simulink model "Full_Car_Model"  (R2023b)
settings: Solver=FixedStepAuto  StartTime=0.0  StopTime=t_end_sim  FixedStep=Ts_sim  RelTol=1e-3
values from neighbouring files (symbols this model uses):
  a_b_ref_sat = [ zeros(1,10) ... (first row only)    [A1_Init.m]    (also in C1_MonteCarloAnalysis.m)
  adaptive = 3    [A1_Init.m]    (also in C1_MonteCarloAnalysis.m = 1)
  data = A2_Full_car_model_parameters_4onBoard()    [A1_Init.m]    (also in C1_MonteCarloAnalysis.m)
  Ft_demand_F = [zeros(1,601) 200*ones(1,2400)]./data.R_F    [A1_Init.m]    (also in C1_MonteCarloAnalysis.m)
  Ft_demand_R = [zeros(1,(601-length(l_discr)))              200*ones(1,(2400+length(l_discr)))]./data.R_R    [A1_Init.m]    (also in C1_MonteCarloAnalysis.m)
  handmade_front = strcat(currentPath,'\Road_profiles\height_crg_files\','handmade_step_3cm_singlefunctions.crg')    [A1_Init.m]    (also in C1_MonteCarloAnalysis.m)
  handmade_mu_front = strcat(currentPath,'\Road_profiles\friction_crg_files\','handmade_fric_step_01_singlefunctions.crg')    [A1_Init.m]    (also in C1_MonteCarloAnalysis.m)
  handmade_mu_rear = handmade_mu_front    [A1_Init.m]    (also in C1_MonteCarloAnalysis.m)
  handmade_rear = handmade_front    [A1_Init.m]    (also in C1_MonteCarloAnalysis.m)
  LowLim_Q1 = -10    [A1_Init.m]    (also in C1_MonteCarloAnalysis.m)
  M = N    (= 10)    [A1_Init.m]    (also in C1_MonteCarloAnalysis.m)
  mu_distance = test_distance    [A1_Init.m]    (also in C1_MonteCarloAnalysis.m)
  mu_road = [ones(1,1001), 0.1*ones(1,2000)]    [A1_Init.m]    (also in C1_MonteCarloAnalysis.m)
  N = 10    [A1_Init.m]    (also in C1_MonteCarloAnalysis.m)
  N_iter = 3    [A1_Init.m]    (also in C1_MonteCarloAnalysis.m)
  omega_ini_F_L = x_u_dot_ini_F_L/data.R_F    [A1_Init.m]    (also in C1_MonteCarloAnalysis.m)
  omega_ini_F_R = x_u_dot_ini_R_R/data.R_F    [A1_Init.m]    (also in C1_MonteCarloAnalysis.m)
  omega_ini_R_L = x_u_dot_ini_R_L/data.R_R +2.483*1e-6    [A1_Init.m]    (also in C1_MonteCarloAnalysis.m)
  omega_ini_R_R = x_u_dot_ini_R_R/data.R_R+2.483*1e-6    [A1_Init.m]    (also in C1_MonteCarloAnalysis.m)
  passive = 2    [A1_Init.m]    (also in C1_MonteCarloAnalysis.m)
  Pitch = 0    [A1_Init.m]    (also in C1_MonteCarloAnalysis.m)
  Pitch_dot = 0    [A1_Init.m]    (also in C1_MonteCarloAnalysis.m)
  preview = 2    [A1_Init.m]    (also in C1_MonteCarloAnalysis.m)
  Q1 = 1e6    (= 1000000)    [A1_Init.m]    (also in C1_MonteCarloAnalysis.m)
  Q1_sat = 0    [A1_Init.m]    (also in C1_MonteCarloAnalysis.m)
  Q2 = 1e5    (= 100000)    [A1_Init.m]    (also in C1_MonteCarloAnalysis.m)
  QN1 = 0    [A1_Init.m]    (also in C1_MonteCarloAnalysis.m)
  QN2 = 0    [A1_Init.m]    (also in C1_MonteCarloAnalysis.m)
  R1 = 1e10    (= 10000000000)    [A1_Init.m]    (also in C1_MonteCarloAnalysis.m)
  r1_h0 = 0.99    [A1_Init.m]    (also in C1_MonteCarloAnalysis.m)
  r1_k = 1000    [A1_Init.m]    (also in C1_MonteCarloAnalysis.m)
  r1_max = 11    [A1_Init.m]    (also in C1_MonteCarloAnalysis.m)
  r1_min = -10    [A1_Init.m]    (also in C1_MonteCarloAnalysis.m)
  r2 = 2    [A1_Init.m]    (also in C1_MonteCarloAnalysis.m)
  R2 = 1e2    (= 100)    [A1_Init.m]    (also in C1_MonteCarloAnalysis.m)
  R2_rl = 2    [A1_Init.m]    (also in C1_MonteCarloAnalysis.m)
  road_profile = [zeros(1,801),ones(1,2200)*10*Step_selector]    [A1_Init.m]    (also in C1_MonteCarloAnalysis.m)
  T_distance = test_distance    [A1_Init.m]    (also in C1_MonteCarloAnalysis.m)
  T_hs_ini_F_L = 0    [A1_Init.m]    (also in C1_MonteCarloAnalysis.m)
  T_hs_ini_F_R = 0    [A1_Init.m]    (also in C1_MonteCarloAnalysis.m)
  T_hs_ini_R_L = 0    [A1_Init.m]    (also in C1_MonteCarloAnalysis.m)
  T_hs_ini_R_R = 0    [A1_Init.m]    (also in C1_MonteCarloAnalysis.m)
  test_distance = 0:0.01:30    [A1_Init.m]    (also in C1_MonteCarloAnalysis.m)
  theta_s_ini_F_L = 0    [A1_Init.m]    (also in C1_MonteCarloAnalysis.m)
  theta_s_ini_F_R = 0    [A1_Init.m]    (also in C1_MonteCarloAnalysis.m)
  theta_s_ini_R_L = 0    [A1_Init.m]    (also in C1_MonteCarloAnalysis.m)
  theta_s_ini_R_R = 0    [A1_Init.m]    (also in C1_MonteCarloAnalysis.m)
  theta_w_ini_F_L = -1.056*1e-2    (= -0.01056)    [A1_Init.m]    (also in C1_MonteCarloAnalysis.m)
  theta_w_ini_R_L = -1.056*1e-2    (= -0.01056)    [A1_Init.m]    (also in C1_MonteCarloAnalysis.m)
  Ts = 1e-3*[0 5 10 15 20 25 30 40 60 80 100]    [A1_Init.m]    (also in C1_MonteCarloAnalysis.m)
  w1_h0 = 0.0008    [A1_Init.m]    (also in C1_MonteCarloAnalysis.m)
  w1_k = 5000    [A1_Init.m]    (also in C1_MonteCarloAnalysis.m)
  w1_max = 9    [A1_Init.m]    (also in C1_MonteCarloAnalysis.m)
  w1_min = -10    [A1_Init.m]    (also in C1_MonteCarloAnalysis.m)
  w1_sat = 0.085    [A1_Init.m]    (also in C1_MonteCarloAnalysis.m)
  w2_h0 = 2    [A1_Init.m]    (also in C1_MonteCarloAnalysis.m)
  w2_inc = 0.05    [A1_Init.m]    (also in C1_MonteCarloAnalysis.m)
  w2_k = 10    [A1_Init.m]    (also in C1_MonteCarloAnalysis.m)
  w2_max = 5.3    [A1_Init.m]    (also in C1_MonteCarloAnalysis.m)
  w2_min = -10    [A1_Init.m]    (also in C1_MonteCarloAnalysis.m)
  Wmat_NMPC_init = [W(1,:) W(2,:) W(3,:) W(4,:)]    [A1_Init.m]    (also in C1_MonteCarloAnalysis.m)
  WNmat_NMPC_init = [WN(1,:) WN(2,:)]    [A1_Init.m]    (also in C1_MonteCarloAnalysis.m)
  X_0 = [z_b_dot_ini z_b_ini z_u_dot_ini_F_L z_u_ini_F_L x_b_dot_ini x_b_ini x_u_dot_ini_F_L x_u_ini_F_L          omega_ini_F_L theta_w_ini_F_L omega_ini_F_L theta_s_ini_F_L torque_ini_F_L]    [A1_Init.m]    (also in C1_MonteCarloAnalysis.m)
  x_b_dot_ini = speed_ini/3.6    (= 11.1111111111)    [A1_Init.m]    (also in C1_MonteCarloAnalysis.m)
  x_b_ini = data.b+pos_ini    [A1_Init.m]    (also in C1_MonteCarloAnalysis.m)
  x_u_dot_ini_F_L = speed_ini/3.6 - 1.125*1e-4    (= 11.1109986111)    [A1_Init.m]    (also in C1_MonteCarloAnalysis.m)
  x_u_dot_ini_F_R = speed_ini/3.6 - 1.125*1e-4    (= 11.1109986111)    [A1_Init.m]    (also in C1_MonteCarloAnalysis.m)
  x_u_dot_ini_R_L = speed_ini/3.6 - 1.125*1e-4    (= 11.1109986111)    [A1_Init.m]    (also in C1_MonteCarloAnalysis.m)
  x_u_dot_ini_R_R = speed_ini/3.6 - 1.125*1e-4    (= 11.1109986111)    [A1_Init.m]    (also in C1_MonteCarloAnalysis.m)
  x_u_ini_F_L = data.a+data.b+pos_ini    [A1_Init.m]    (also in C1_MonteCarloAnalysis.m)
  x_u_ini_F_R = data.a+data.b+pos_ini    [A1_Init.m]    (also in C1_MonteCarloAnalysis.m)
  x_u_ini_R_L = pos_ini    (= 0)    [A1_Init.m]    (also in C1_MonteCarloAnalysis.m)
  x_u_ini_R_R = pos_ini    (= 0)    [A1_Init.m]    (also in C1_MonteCarloAnalysis.m)
  z_b_dot_ini = 0    [A1_Init.m]    (also in C1_MonteCarloAnalysis.m)
  z_b_ini = 0    [A1_Init.m]    (also in C1_MonteCarloAnalysis.m)
  z_u_dot_ini_F_L = 0    [A1_Init.m]    (also in C1_MonteCarloAnalysis.m)
  z_u_dot_ini_F_R = 0    [A1_Init.m]    (also in C1_MonteCarloAnalysis.m)
  z_u_dot_ini_R_L = 0    [A1_Init.m]    (also in C1_MonteCarloAnalysis.m)
  z_u_dot_ini_R_R = 0    [A1_Init.m]    (also in C1_MonteCarloAnalysis.m)
  z_u_ini_F_L = 0    [A1_Init.m]    (also in C1_MonteCarloAnalysis.m)
  z_u_ini_F_R = 0    [A1_Init.m]    (also in C1_MonteCarloAnalysis.m)
  z_u_ini_R_L = 0    [A1_Init.m]    (also in C1_MonteCarloAnalysis.m)
  z_u_ini_R_R = 0    [A1_Init.m]    (also in C1_MonteCarloAnalysis.m)
undefined symbols (not defined in the file or in its folder): Delay_step, road_with_noise
libraries: mfswift_library x8, rllib x4, simulink x4
(part 7 of 7)

== matlab function Full_Car_Model/CONTROLLER REAR LEFT/Rule based/MATLAB Function3 ==
  data: flag input; mu_prev input; W output; M parameter; r1_min parameter; r1_max parameter; r1_k parameter; r1_h0 parameter
function W = fcn(flag, mu_prev,M, r1_min, r1_max, r1_k, r1_h0)
h=0; 

x2 = linspace(0, 1, M+1);    
exp_growth = exp(1 * x2) - 1;  

perc = exp_growth; 
perc = perc / sum(perc);

for i=1:M+1
    h=h+mu_prev(i)*perc(i);
end

W=r1_min+(r1_max-r1_min)/(1+exp(r1_k*(abs(h)-r1_h0)));

if not(flag)
    W = r1_min;
end

== matlab function Full_Car_Model/PLANT MODEL WITH MF-SWIFT/4 ON-BOARD POWERTRAIN - FRONT/LEFT HALF SHAFT TORQUES WITH BACKLASH/MATLAB Function2 ==
  data: f1 output; delta_theta input; backlash_F4 input
function f1 = f1_with_backlash(delta_theta, backlash_F4)

if delta_theta < -backlash_F4
    f1 = 1;
else
    f1 = 0;
end

== matlab function Full_Car_Model/PLANT MODEL WITH MF-SWIFT/4 ON-BOARD POWERTRAIN - FRONT/LEFT HALF SHAFT TORQUES WITH BACKLASH/MATLAB Function3 ==
  data: f2 output; delta_theta input; backlash_F4 input
function f2 = f2_with_backlash(delta_theta, backlash_F4)

if delta_theta > backlash_F4
    f2 = 1;
else
    f2 = 0;
end

== matlab function Full_Car_Model/PLANT MODEL WITH MF-SWIFT/4 ON-BOARD POWERTRAIN - FRONT/SHAFT EQUATIONS ==
  data: theta_s_ddot_L output; T_t_L input; theta_s_ddot_R output; T_hs_L input; T_t_R input; T_hs_R input; data parameter
function [theta_s_ddot_L, theta_s_ddot_R] = open_differential_equations(T_t_L, T_hs_L, T_t_R, T_hs_R, data)

theta_s_ddot_L = (T_t_L - T_hs_L) / data.J_eq_F4;
theta_s_ddot_R = (T_t_R - T_hs_R) / data.J_eq_F4;

== matlab function Full_Car_Model/PLANT MODEL WITH MF-SWIFT/4 ON-BOARD POWERTRAIN - FRONT/RIGHT HALF SHAFT TORQUES WITH BACKLASH/MATLAB Function2 ==
  data: f1 output; delta_theta input; backlash_F4 input
function f1 = f1_with_backlash(delta_theta, backlash_F4)

if delta_theta < -backlash_F4
    f1 = 1;
else
    f1 = 0;
end

== matlab function Full_Car_Model/PLANT MODEL WITH MF-SWIFT/4 ON-BOARD POWERTRAIN - FRONT/RIGHT HALF SHAFT TORQUES WITH BACKLASH/MATLAB Function3 ==
  data: f2 output; delta_theta input; backlash_F4 input
function f2 = f2_with_backlash(delta_theta, backlash_F4)

if delta_theta > backlash_F4
    f2 = 1;
else
    f2 = 0;
end

== matlab function Full_Car_Model/PLANT MODEL WITH MF-SWIFT/4 ON-BOARD POWERTRAIN - REAR/LEFT HALF SHAFT TORQUES WITH BACKLASH/MATLAB Function2 ==
  data: f1 output; delta_theta input; backlash_R4 input
function f1 = f1_with_backlash(delta_theta, backlash_R4)

if delta_theta < -backlash_R4
    f1 = 1;
else
    f1 = 0;
end

== matlab function Full_Car_Model/PLANT MODEL WITH MF-SWIFT/4 ON-BOARD POWERTRAIN - REAR/LEFT HALF SHAFT TORQUES WITH BACKLASH/MATLAB Function3 ==
  data: f2 output; delta_theta input; backlash_R4 input
function f2 = f2_with_backlash(delta_theta, backlash_R4)

if delta_theta > backlash_R4
    f2 = 1;
else
    f2 = 0;
end

== matlab function Full_Car_Model/PLANT MODEL WITH MF-SWIFT/4 ON-BOARD POWERTRAIN - REAR/OPEN DIFFERENTIAL EQUATIONS ==
  data: theta_s_ddot_L output; T_t_L input; theta_s_ddot_R output; T_hs_L input; T_t_R input; T_hs_R input; data parameter
function [theta_s_ddot_L, theta_s_ddot_R] = open_differential_equations(T_t_L, T_hs_L, T_t_R, T_hs_R, data)

theta_s_ddot_L = (T_t_L - T_hs_L) / data.J_eq_R4;
theta_s_ddot_R = (T_t_R - T_hs_R) / data.J_eq_R4;

== matlab function Full_Car_Model/PLANT MODEL WITH MF-SWIFT/4 ON-BOARD POWERTRAIN - REAR/RIGHT HALF SHAFT TORQUES WITH BACKLASH/MATLAB Function2 ==
  data: f1 output; delta_theta input; backlash_R4 input
function f1 = f1_with_backlash(delta_theta, backlash_R4)

if delta_theta < -backlash_R4
    f1 = 1;
else
    f1 = 0;
end

== matlab function Full_Car_Model/PLANT MODEL WITH MF-SWIFT/4 ON-BOARD POWERTRAIN - REAR/RIGHT HALF SHAFT TORQUES WITH BACKLASH/MATLAB Function3 ==
  data: f2 output; delta_theta input; backlash_R4 input
function f2 = f2_with_backlash(delta_theta, backlash_R4)

if delta_theta > backlash_R4
    f2 = 1;
else
    f2 = 0;
end

== matlab function Full_Car_Model/PLANT MODEL WITH MF-SWIFT/SUSPENSION MODEL/LONGITUDINAL DYNAMICS/Longitudinal Balance ==
  data: x_b_dot input; Fk_x_R_L input; Fc_x_R_L input; Fk_x_R_R input; Fc_x_R_R input; Fk_x_F_L input; Fc_x_F_L input; Fk_x_F_R input; Fc_x_F_R input; F_x_R_L input; F_x_R_R input; F_x_F_L input; F_x_F_R input; x_b_dot_dot output; x_u_dot_dot_R_L output; x_u_dot_dot_R_R output; x_u_dot_dot_F_L output; x_u_dot_dot_F_R output; data parameter
function [x_b_dot_dot, x_u_dot_dot_R_L, x_u_dot_dot_R_R, x_u_dot_dot_F_L, x_u_dot_dot_F_R] = ...
    fcn(x_b_dot, Fk_x_R_L, Fc_x_R_L, Fk_x_R_R, Fc_x_R_R, Fk_x_F_L, Fc_x_F_L, Fk_x_F_R, Fc_x_F_R, F_x_R_L, F_x_R_R, F_x_F_L, F_x_F_R, data)

F_drag = data.Aero_Coeff*x_b_dot^2;

x_b_dot_dot = (- Fk_x_R_L - Fc_x_R_L - Fk_x_R_R - Fc_x_R_R...
               - Fk_x_F_L - Fc_x_F_L - Fk_x_F_R - Fc_x_F_R...
               - F_drag) / data.m_b;
x_u_dot_dot_R_L = (Fk_x_R_L + Fc_x_R_L + F_x_R_L) / data.m_u_R;
x_u_dot_dot_R_R = (Fk_x_R_R + Fc_x_R_R + F_x_R_R) / data.m_u_R;

x_u_dot_dot_F_L = (Fk_x_F_L + Fc_x_F_L + F_x_F_L) / data.m_u_F;
x_u_dot_dot_F_R = (Fk_x_F_R + Fc_x_F_R + F_x_F_R) / data.m_u_F;

== matlab function Full_Car_Model/CONTROLLER FRONT RIGHT/RL_weights/MATLAB Function ==
  data: w_prev input; h output; M parameter
function h = fcn(w_prev,M)
h=0;   
w1_memo=5;
w_var=zeros(1,M+w1_memo+1);

x1 = linspace(0, 1, w1_memo);         
x2 = linspace(1, 0, M+1); 
exp_growth = exp(1 * x1) - 1;   
exp_decay = exp(1 * x2) - 1;  

perc = [exp_growth, exp_decay]; 
perc = perc / sum(perc);

for i=1:M+w1_memo
    w_var(i)=w_prev(i+1)-w_prev(i); 
    h=h+w_var(i)*perc(i);
end

== matlab function Full_Car_Model/PLANT MODEL WITH MF-SWIFT/SUSPENSION MODEL/ROTATIONAL DYNAMICS/Angular balance ==
  data: Fk_x_R_L input; Fc_x_R_L input; Fk_z_R_L input; Fc_z_R_L input; Fk_x_R_R input; Fc_x_R_R input; Fk_z_R_R input; Fc_z_R_R input; Fk_x_F_L input; Fc_x_F_L input; Fk_z_F_L input; Fc_z_F_L input; Fk_x_F_R input; Fc_x_F_R input; Fk_z_F_R input; Fc_z_F_R input; Mz_AP input; Fu_z_R_L input; Fu_z_R_R input; Fu_z_F_L input; Fu_z_F_R input; pitch_dot_dot output; data parameter
function pitch_dot_dot  ...
    = fcn(Fk_x_R_L, Fc_x_R_L, Fk_z_R_L, Fc_z_R_L, Fk_x_R_R, Fc_x_R_R, Fk_z_R_R, Fc_z_R_R,...
    Fk_x_F_L, Fc_x_F_L, Fk_z_F_L, Fc_z_F_L, Fk_x_F_R, Fc_x_F_R, Fk_z_F_R, Fc_z_F_R,...
    Mz_AP, Fu_z_R_L, Fu_z_R_R, Fu_z_F_L, Fu_z_F_R, data)

pitch_dot_dot = ( (Fk_z_R_L + Fc_z_R_L + Fu_z_R_L + Fk_z_R_R + Fc_z_R_R + Fu_z_R_R)*data.b...
                 -(Fk_z_F_L + Fc_z_F_L + Fu_z_F_L + Fk_z_F_R + Fc_z_F_R + Fu_z_F_R)*data.a...
                 -(Fk_x_R_L + Fc_x_R_L + Fk_x_R_R + Fc_x_R_R + Fk_x_F_L + Fc_x_F_L + Fk_x_F_R + Fc_x_F_R)*data.hg...
                 + Mz_AP)/ (2*data.I_b_y);

== matlab function Full_Car_Model/PLANT MODEL WITH MF-SWIFT/SUSPENSION MODEL/VERTICAL DYNAMICS/Vertical Balance ==
  data: z_b_dot_dot output; z_u_dot_dot_R_L output; z_u_dot_dot_R_R output; Fk_z_R_L input; Fc_z_R_L input; Fk_z_R_R input; Fc_z_R_R input; Fk_z_F_L input; Fc_z_F_L input; Fk_z_F_R input; Fc_z_F_R input; F_z_R_L input; F_z_R_R input; F_z_F_L input; F_z_F_R input; Fu_AP_F input; Fu_AP_R input; Fz_AP input; Fu_z_R_L input; Fu_z_R_R input; Fu_z_F_L input; Fu_z_F_R input; z_u_dot_dot_F_L output; z_u_dot_dot_F_R output; data parameter
function [z_b_dot_dot, z_u_dot_dot_R_L, z_u_dot_dot_R_R, z_u_dot_dot_F_L, z_u_dot_dot_F_R] =...
    fcn(Fk_z_R_L, Fc_z_R_L, Fk_z_R_R, Fc_z_R_R, Fk_z_F_L, Fc_z_F_L, Fk_z_F_R, Fc_z_F_R,...
    F_z_R_L, F_z_R_R, F_z_F_L, F_z_F_R, Fu_AP_F, Fu_AP_R, Fz_AP,...
    Fu_z_R_L, Fu_z_R_R, Fu_z_F_L, Fu_z_F_R, data)

z_b_dot_dot = (- Fk_z_R_L - Fk_z_R_R - Fk_z_F_L - Fk_z_F_R...
               - Fc_z_R_L - Fc_z_R_R - Fc_z_F_L - Fc_z_F_R...
               - Fu_z_R_L - Fu_z_R_R - Fu_z_F_L - Fu_z_F_R...
               + Fz_AP) / data.m_b;
           
z_u_dot_dot_R_L  = (Fk_z_R_L + Fc_z_R_L + F_z_R_L + Fu_z_R_L - Fu_AP_R) / data.m_u_R;
z_u_dot_dot_R_R  = (Fk_z_R_R + Fc_z_R_R + F_z_R_R + Fu_z_R_R - Fu_AP_R) / data.m_u_R;

z_u_dot_dot_F_L  = (Fk_z_F_L + Fc_z_F_L + F_z_F_L + Fu_z_F_L - Fu_AP_F) / data.m_u_F;
z_u_dot_dot_F_R  = (Fk_z_F_R + Fc_z_F_R + F_z_F_R + Fu_z_F_R - Fu_AP_F) / data.m_u_F;

== matlab function Full_Car_Model/CONTROLLER FRONT LEFT/MATLAB Function ==
  data: z_b_dot input; z_b_dot_F output; z_b input; z_u_dot_F_L input; z_u_F_L input; x_b_dot input; x_b input; x_u_dot_F_L input; x_u_F_L input; theta_w_dot input; theta_w input; theta_s_dot input; theta_s input; z_b_F output; z_u_dot_F_L output; z_u_F_L output; x_b_dot_F output; x_b_F output; x_u_dot_F_L output; x_u_F_L output; theta_w_dot output; theta_w output; theta_s_dot output; theta_s output; torque input; torque output; pitch_dot input; pitch input; a input
function [z_b_dot_F, z_b_F, z_u_dot_F_L, z_u_F_L,...
          x_b_dot_F, x_b_F, x_u_dot_F_L, x_u_F_L,...
          theta_w_dot, theta_w, theta_s_dot, theta_s, torque]...
          = fcn(z_b_dot, z_b, z_u_dot_F_L, z_u_F_L,...
                x_b_dot, x_b, x_u_dot_F_L, x_u_F_L,...
                theta_w_dot, theta_w, theta_s_dot, theta_s, torque,...
                pitch_dot, pitch, a)

z_b_dot_F   = z_b_dot + pitch_dot*a;
z_b_F       = z_b + a*tan(pitch);
x_b_dot_F   = x_b_dot;
x_b_F       = x_b + a;

end

== matlab function Full_Car_Model/CONTROLLER FRONT LEFT/RL_weights/MATLAB Function ==
  data: w_prev input; h output; M parameter
function h = fcn(w_prev,M)
h=0;   
w1_memo=5;
w_var=zeros(1,M+w1_memo+1);

x1 = linspace(0, 1, w1_memo);         
x2 = linspace(1, 0, M+1); 
exp_growth = exp(1 * x1) - 1;   
exp_decay = exp(1 * x2) - 1;  

perc = [exp_growth, exp_decay]; 
perc = perc / sum(perc);

for i=1:M+w1_memo
    w_var(i)=w_prev(i+1)-w_prev(i); 
    h=h+w_var(i)*perc(i);
end

== matlab function Full_Car_Model/CONTROLLER FRONT RIGHT/Reference acceleration/a_b_ref ==
  data: Ft input; vCar_k input; data parameter; a_b_ref output
function a_b_ref    = fcn(Ft, vCar_k, data)

I_y         = data.I_y_F;
rho_air     = data.rho_air;
C_d         = data.C_d;
A_car       = data.A_car;

m_total     = data.m_total;
f_0         = data.f_0_F;

f_2         = data.f_2_F;
f           = f_0 + f_2*vCar_k^2;

a_b_ref     = (2*Ft*data.i_t_F4*data.n_t_F4 - 0.5*rho_air*C_d*A_car*vCar_k^2 - f*m_total*data.g)/(m_total + 4*I_y/(data.R_F^2)); %1\ 0.374 2\ 0.179
end

== matlab function Full_Car_Model/CONTROLLER REAR LEFT/Reference Generation ==
  data: a_b_ref input; References output; N parameter; data parameter
function References    = fcn(a_b_ref, N, data)

 href=[a_b_ref 0 0 0];                      
 References_horizon = [repmat(href,N,1)].';
 hN = [a_b_ref 0];
 References_end = hN.';

References=[References_horizon(:); References_end(:)];
end

== matlab function Full_Car_Model/CONTROLLER REAR RIGHT/Reference Generation ==
  data: a_b_ref input; References output; N parameter; data parameter
function References    = fcn(a_b_ref, N, data)

 href=[a_b_ref 0 0 0];                      
 References_horizon = [repmat(href,N,1)].';
 hN = [a_b_ref 0];
 References_end = hN.';

References=[References_horizon(:); References_end(:)];
end

== matlab function Full_Car_Model/CONTROLLER REAR LEFT/Reference acceleration/a_b_ref ==
  data: Ft input; vCar_k input; data parameter; a_b_ref output
function a_b_ref    = fcn(Ft, vCar_k, data)

I_y         = data.I_y_F;
rho_air     = data.rho_air;
C_d         = data.C_d;
A_car       = data.A_car;

m_total     = data.m_total;
f_0         = data.f_0_F;

f_2         = data.f_2_F;
f           = f_0 + f_2*vCar_k^2;

a_b_ref     = (2*Ft*data.i_t_F4*data.n_t_F4 - 0.5*rho_air*C_d*A_car*vCar_k^2 - f*m_total*data.g)/(m_total + 4*I_y/(data.R_F^2)); %1\ 0.374 2\ 0.179
end

== matlab function Full_Car_Model/CONTROLLER REAR RIGHT/Reference acceleration/a_b_ref ==
  data: Ft input; vCar_k input; data parameter; a_b_ref output
function a_b_ref    = fcn(Ft, vCar_k, data)

I_y         = data.I_y_F;
rho_air     = data.rho_air;
C_d         = data.C_d;
A_car       = data.A_car;

m_total     = data.m_total;
f_0         = data.f_0_F;

f_2         = data.f_2_F;
f           = f_0 + f_2*vCar_k^2;

a_b_ref     = (2*Ft*data.i_t_F4*data.n_t_F4 - 0.5*rho_air*C_d*A_car*vCar_k^2 - f*m_total*data.g)/(m_total + 4*I_y/(data.R_F^2)); %1\ 0.374 2\ 0.179
end

== matlab function Full_Car_Model/CONTROLLER FRONT LEFT/Reference acceleration/a_b_ref ==
  data: Ft input; vCar_k input; data parameter; a_b_ref output
function a_b_ref    = fcn(Ft, vCar_k, data)

I_y         = data.I_y_F;
rho_air     = data.rho_air;
C_d         = data.C_d;
A_car       = data.A_car;

m_total     = data.m_total;
f_0         = data.f_0_F;

f_2         = data.f_2_F;
f           = f_0 + f_2*vCar_k^2;

a_b_ref     = (2*Ft*data.i_t_F4*data.n_t_F4 - 0.5*rho_air*C_d*A_car*vCar_k^2 - f*m_total*data.g)/(m_total + 4*I_y/(data.R_F^2)); %1\ 0.374 2\ 0.179
end

== matlab function Full_Car_Model/CONTROLLER FRONT RIGHT/RL_weights/MATLAB Function3 ==
  data: mu_prev input; h output; M parameter
function h = fcn(mu_prev,M)
h=0; 

x2 = linspace(1, 0, M+1);    
exp_decay = exp(1 * x2) - 1;  

perc = exp_decay; 
perc = perc / sum(perc);

for i=1:M+1
    h=h+mu_prev(i)*perc(i);
end

== matlab function Full_Car_Model/CONTROLLER FRONT LEFT/ROAD PREVIEW/NO_ROAD_PREVIEW ==
  data: w input; OnlineData output; Tm_req input; Tm_req_F2 input; Tm_req_R_L input; Tm_req_R_R input; N parameter; mu_act input; sigma_ref input
function OnlineData=OnlineDataArray(w, Tm_req, Tm_req_F2, Tm_req_R_L, Tm_req_R_R, N, mu_act, sigma_ref)

OnlineData = repmat([w; 0; Tm_req; Tm_req_F2; Tm_req_R_L; Tm_req_R_R; mu_act; sigma_ref],N+1,1);
end

== matlab function Full_Car_Model/CONTROLLER REAR RIGHT/MATLAB Function ==
  data: z_b_dot input; z_b_dot_R output; z_b input; z_u_dot_R_R input; z_u_R_R input; x_b_dot input; x_b input; x_u_dot_R_R input; x_u_R_R input; theta_w_dot input; theta_w input; theta_s_dot input; theta_s input; z_b_R output; z_u_dot_R_R output; z_u_R_R output; x_b_dot_R output; x_b_R output; x_u_dot_R_R output; x_u_R_R output; theta_w_dot output; theta_w output; theta_s_dot output; theta_s output; torque input; torque output; pitch_dot input; pitch input; b input
function [z_b_dot_R, z_b_R, z_u_dot_R_R, z_u_R_R,...
          x_b_dot_R, x_b_R, x_u_dot_R_R, x_u_R_R,...
          theta_w_dot, theta_w, theta_s_dot, theta_s, torque]...
          = fcn(z_b_dot, z_b, z_u_dot_R_R, z_u_R_R,...
                x_b_dot, x_b, x_u_dot_R_R, x_u_R_R,...
                theta_w_dot, theta_w, theta_s_dot, theta_s, torque,...
                pitch_dot, pitch, b)

z_b_dot_R   = z_b_dot - pitch_dot*b;
z_b_R       = z_b - b*pitch;
x_b_dot_R   = x_b_dot;
x_b_R       = x_b - b;

end
